simulink model "SD_Datalogger2"  (Simulink 7.7)
settings: Solver=FixedStepDiscrete  StartTime=0.0  StopTime=10.0  FixedStep=0.001  RelTol=1e-3
libraries: dsPICdrivers x3
settings Model: Creator=ij8977  LastModifiedBy=ij8977
settings OptimizationCC: OptimizeModelRefInitCode=on  LifeSpan=1
settings RTWCC: SystemTargetFile=pic32.tlc  MakeCommand=make_CreateMPLAB  TemplateMakefile=pic32_gcc.tmf  PostCodeGenCommand=dsPIC_Compile()  Description=Embedded Target for Microchip dsPIC (real-time)  ProcessScript=pic32_make_rtw_hook
settings CodeAppCC: IgnoreCustomStorageClasses=off
settings STFCustomTargetCC: FunctionExecutionProfile=off  IncludeMdlTerminateFcn=off  CombineOutputUpdateFcns=on  SuppressErrorStatus=on  ERTCustomFileBanners=on  SupportContinuousTime=off  SupportNonInlinedSFcns=off  SystemTargetFile=pic32.tlc
settings ERTTargetCC: FunctionExecutionProfile=off  MultiwordLength=2048  ParMdlRefBuildCompliant=off  CompOptLevelCompliant=off  IncludeMdlTerminateFcn=off  SuppressErrorStatus=on  ERTFirstTimeCompliant=off  ModelStepFunctionPrototypeControlCompliant=off  CPPClassGenCompliant=off  InlinedParameterPlacement=NonHierarchical  ERTSrcFileBannerTemplate=dsPIC_code_template.cgt  ERTHdrFileBannerTemplate=dsPIC_code_template.cgt  ERTDataSrcFileTemplate=dsPIC_code_template.cgt  ERTDataHdrFileTemplate=dsPIC_code_template.cgt  ERTCustomFileTemplate=dsPIC_main.tlc  ConvertIfToSwitch=off
settings CustomProperty: DataType=string  Value=C:\PROGRA~1\MATLAB\R2011a\bin\win32\gmake

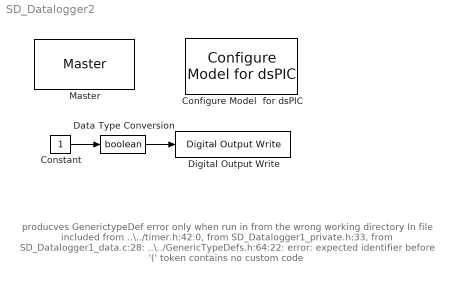
== system SD_Datalogger2 ==
  note: producves GenerictypeDef error only when run in from the wrong working directory
      | In file included from ..\../timer.h:42:0,
      |                  from SD_Datalogger1_private.h:33,
      |                  from SD_Datalogger1_data.c:28:
      | ..\../GenericTypeDefs.h:64:22: error: expected identifier before '(' token
      |
      | contains no custom code
  Configure Model  for dsPIC : dsPICdrivers/Simulink Configuration/Configure Model  for dsPIC
  Constant : Constant
  Data Type Conversion : DataTypeConversion  OutDataTypeStr=boolean
  Digital Output Write : dsPICdrivers/Digital I//O/Digital Output Write  Tag=dsPIC_Digital_Output  Priority=5  PORT=F  Pin=[2]  Simultaneous=off  OrderingInOutPopup=None
  Master : dsPICdrivers/Master  Tag=dsPIC_MASTER  Priority=1  TimeStepType=Timer1  picType=32MX460F512L  fcy=40000000  Quartz_33f=8e6  PLLActive_33f=on  fcyDesired_33f=40e6  tmr1="[1  39999  0]"  tmr1Info="Time Step : 0.001  ;   Error : 0%  PR1=39999"  tmr2345="[0  0  0  0]"  tmr2345cfg=[-1 -1 -1 -1]  IOautoConf=on  typePort="[ 0   0   0   0   0   0   0   0   0   0   0   0   0   0   0   0   0   0   0   0   0   0   0   0   0   0   0   0   0   0   0   0   0   0   0   0   0   0   0   0   0   0   0   0   0   0   0   0   0   0   0   0   0   0   0   0   0   0   0   0   0   0   0   0   0   0   0   0   0   0   0   0   0   0   0   0   0   0   0   0   0   0  10   0   0   0   0   0   0   0   0   0   0   0   0   0   0   0   0   0   0   0   0   0   0   0   0   0   0   0   0   0 ]"  TRIS="[ 65535  65535  65535  65535  65535  65531  65535 ]"  ADPCFG=0  MasterBusyPort=None  MasterOverloadPort=None  FOSC=Quartz (XT - HS)  ClockSwitchMonitor=Both disabled  TempProtection_33f=TEMP_ON  FPBOR=<empty>  PWRT=disable  MCLR=<empty>  ICD=ICS_PGD1  JTAGEN=JTAGEN_OFF  PowerSave=off  OverrideFcy=off  NewFcy=1e6  PR2345="[65535  65535  65535  65535]"
  wires:
  Constant/1 -> Data Type Conversion/1
  Data Type Conversion/1 -> Digital Output Write/1
